simulink model "simulink6"  (R2026b)
settings: Solver=ode113  StopTime=20.0  FixedStep=0.0001
values from neighbouring files (symbols this model uses):
  A = [0 0 1 0 ... (first row only)    [QUBE2_ROTPEN_ABCD_eqns.m]
  B = kt * B / Rm    [QUBE2_ROTPEN_ABCD_eqns.m]
  C = eye(4,4)    [QUBE2_ROTPEN_ABCD_eqns.m]
  D = zeros(4,1)    [QUBE2_ROTPEN_ABCD_eqns.m]
  K = lqr(A, B, Q, R)    [setup_qube2_rotpen_wo_input.m]
  kr = [0; 0; 0; 0]    [setup_qube2_rotpen_wo_input.m]
  x0 = [1; 0; 0; 0]    [setup_qube2_rotpen_wo_input.m]
settings Model: Creator=leelou  LastModifiedBy=leelou

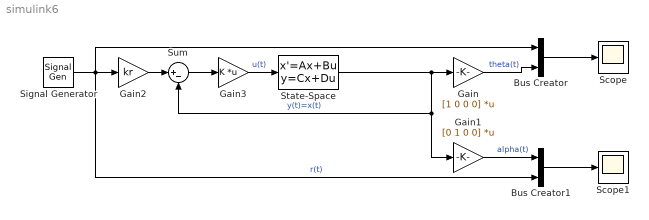
== system simulink6 ==
  Bus Creator : BusCreator  Inputs=2
  Bus Creator1 : BusCreator  Inputs=2
  Gain : Gain  Gain=[1 0 0 0]  Multiplication=Matrix(K*u) (u vector)
  Gain1 : Gain  Gain=[0 1 0 0]  Multiplication=Matrix(K*u) (u vector)
  Gain2 : Gain  Gain=kr
  Gain3 : Gain  Gain=K  Multiplication=Matrix(K*u) (u vector)
  Scope : Scope
      settings: ActiveDisplayYMinimum=-1.25  ActiveDisplayYMaximum=1.25
  Scope1 : Scope
      settings: ActiveDisplayYMinimum=-1.25  ActiveDisplayYMaximum=1.25
  Signal Generator : SignalGenerator  WaveForm=square  Frequency=0.125
  State-Space : StateSpace  A=A  B=B  C=C  D=D  InitialCondition=x0
  Sum : Sum  Inputs=|+-
  wires:
  Bus Creator/1 -> Scope/1
  Bus Creator1/1 -> Scope1/1
  Gain1/1 -> Bus Creator1/1  "alpha(t)"
  State-Space/1 -> Gain1/1, Sum/2, Gain/1  "y(t)=x(t)"
  Signal Generator/1 -> Bus Creator1/2, Bus Creator/1, Gain2/1  "r(t)"
  Gain2/1 -> Sum/1
  Gain/1 -> Bus Creator/2  "theta(t)"
  Gain3/1 -> State-Space/1  "u(t)"
  Sum/1 -> Gain3/1
